simulink model "s_c_nbe_m32k"  (R2018a)
settings: Solver=VariableStepDiscrete  StartTime=0.0  StopTime=1000  RelTol=1e-3
undefined symbols (not defined in the file): fft_stages, n_taps, output_bits, pfb_coeff_gen_calc, xengbits
libraries: xbsIndex_r4 x23714, casper_library_misc x17, xps_library x4, casper_library_scopes x4, xbsReplacements_r4 x4
(part 120 of 171)

== system s_c_nbe_m32k/nb_pfb/pfb_fir_generic1/pfb_fir_coeff_gen/b_expand ==
  bus_in : Inport
  reinterpret1 : xbsIndex_r4/Reinterpret  force_arith_type=on  arith_type=Unsigned  force_bin_pt=on  bin_pt=0  block_type=reinterpret
  reinterpret2 : xbsIndex_r4/Reinterpret  force_arith_type=on  arith_type=Unsigned  force_bin_pt=on  bin_pt=0  block_type=reinterpret
  slice1 : xbsIndex_r4/Slice  nbits=18  boolean_output=off  mode=Upper Bit Location + Width  bit1=-18  base1=MSB of Input  bit0=0  base0=LSB of Input  dbl_ovrd=off  block_type=slice
  slice2 : xbsIndex_r4/Slice  nbits=18  boolean_output=off  mode=Upper Bit Location + Width  bit1=0  base1=MSB of Input  bit0=0  base0=LSB of Input  dbl_ovrd=off  block_type=slice
  msb_out2 : Outport
  lsb_out1 : Outport  Port=2
  wires:
  bus_in/1 -> slice2/1, slice1/1
  slice2/1 -> reinterpret2/1
  reinterpret2/1 -> msb_out2/1
  slice1/1 -> reinterpret1/1
  reinterpret1/1 -> lsb_out1/1

== system s_c_nbe_m32k/nb_pfb/pfb_fir_generic1/pfb_fir_coeff_gen/munge ==
  din : Inport
  join : Subsystem  AncestorBlock=casper_library_flow_control/bus_create  mask(bus_create){inputNum=2}
      mask prompts: inputNum "Number of inputs:"
      mask init:
      | bus_create_init(gcb,...
      |     'inputNum', inputNum);
  reinterpret : xbsIndex_r4/Reinterpret  force_arith_type=on  arith_type=Unsigned  force_bin_pt=on  bin_pt=0  block_type=reinterpret
  reinterpret_out : xbsIndex_r4/Reinterpret  force_arith_type=on  arith_type=Unsigned  force_bin_pt=on  bin_pt=0  block_type=reinterpret
  split : Subsystem  AncestorBlock=casper_library_flow_control/bus_expand  mask(bus_expand){mode=divisions of arbitrary size, outputNum=1, outputWidth=[18 18], outputBinaryPt=[0 0], outputArithmeticType=[0 0], show_format=off, outputToWorkspace=off, variablePrefix=out, outputToModelAsWell=on}
      mask prompts: outputNum "Number of outputs:"; outputWidth "Output width [msb ... lsb]:"; outputBinaryPt "Output binary point position [msb ... lsb]:"; outputArithmeticType "Output arithmetic type (ufix=0, fix=1, bool=2) [msb ... lsb]:"; show_format "Print format string?"; outputToWorkspace "Output to workspace?"; variablePrefix "Variable name prefix:"; outputToModelAsWell "Output to model as well?"
      mask help:
      | Expands a 'bus' made using a bus_create or Xilinx
      | concat block.
      | The input will be divided into the specified number
      | of outputs with the specified arithmetic types.
      | Divisions are made from most significant bit.
      mask init: same as s_c_nbe_m32k/bus_expand1
      settings: AttributesFormatString=2 outputs
      mask TypeOptions mode: divisions of equal size | divisions of arbitrary size
      mask Callback mode: bus_expand_callback();
      mask Callback outputWidth: bus_expand_callback();
      mask Callback outputToWorkspace: bus_expand_callback();
  dout : Outport
  wires:
  reinterpret_out/1 -> dout/1
  din/1 -> reinterpret/1
  reinterpret/1 -> split/1(bus_in)
  join/1(bus_out) -> reinterpret_out/1
  split/2(lsb_out1) -> join/1(in1)
  split/1(msb_out2) -> join/2(in2)

== system s_c_nbe_m32k/nb_pfb/pfb_fir_generic1/pfb_fir_coeff_gen/rom ==
  addra : Inport
  dina : Inport  Port=2
  wea : Inport  Port=3
  addrb : Inport  Port=4
  dinb : Inport  Port=5
  web : Inport  Port=6
  A_bussify0 : Subsystem  AncestorBlock=casper_library_flow_control/bus_create  mask(bus_create){inputNum=36}
      mask prompts: inputNum "Number of inputs:"
      mask init:
      | bus_create_init(gcb,...
      |     'inputNum', inputNum);
  B_bussify0 : Subsystem  AncestorBlock=casper_library_flow_control/bus_create  mask(bus_create){inputNum=36}
      mask prompts: inputNum "Number of inputs:"
      mask init:
      | bus_create_init(gcb,...
      |     'inputNum', inputNum);
  alsbs_slice : xbsIndex_r4/Slice  nbits=15  boolean_output=off  mode=Lower Bit Location + Width  bit1=0  base1=LSB of Input  bit0=0  base0=LSB of Input  dbl_ovrd=off  block_type=slice
  blsbs_slice : xbsIndex_r4/Slice  nbits=15  boolean_output=off  mode=Lower Bit Location + Width  bit1=0  base1=LSB of Input  bit0=0  base0=LSB of Input  dbl_ovrd=off  block_type=slice
  bram0_{0..35} (36 alike) : xbsIndex_r4/Dual Port RAM  depth=32768  initVector=getfield(get_param(gcb, 'UserData'), 'initVector')  distributed_mem=Block RAM  init_a=0  init_b=0  rst_a=off  rst_b=off  en_a=off  en_b=off  latency=7  write_mode_A=Read Before Write  write_mode_B=Read Before Write  optimize=Speed  dbl_ovrd=off  block_type=dpram
  ddina0 : xbsIndex_r4/Delay  rst=off  infoeditControl=Selection of Reset will increase slice count due to use of real FFs and instead of SRLs  en=off  latency=0  reg_retiming=on  dbl_ovrd=off  block_type=delay
  ddinb0 : xbsIndex_r4/Delay  rst=off  infoeditControl=Selection of Reset will increase slice count due to use of real FFs and instead of SRLs  en=off  latency=0  reg_retiming=on  dbl_ovrd=off  block_type=delay
  debus_addra0 : Subsystem  AncestorBlock=casper_library_flow_control/bus_expand  mask(bus_expand){mode=divisions of equal size, outputNum=36, outputWidth=[15 15 15 15 15 15 15 15 15 15 15 15 15 15 15 15 15 15 15 15 15 15 15 15 15 15 15 15 15 15 15 15 15 15 15 15], outputBinaryPt=[0 0 0 0 0 0 0 0 0 0 0 0 0 0 0 0 0 0 0 0 0 0 0 0 0 0 0 0 0 0 0 0 0 0 0 0], outputArithmeticType=[0 0 0 0 0 0 0 0 0 0 0 0 0 0 0 0 0 0 0 0 0 0 0 0 0 0 0 0 0 0 0 0 0 0 0 0], show_format=on, outputToWorkspace=off, variablePrefix=, outputToModelAsWell=on}
      mask prompts: outputNum "Number of outputs:"; outputWidth "Output width:"; outputBinaryPt "Output binary point position:"; outputArithmeticType "Output arithmetic type (ufix=0, fix=1, bool=2):"; show_format "Print format string?"; outputToWorkspace "Output to workspace?"; variablePrefix "Variable name prefix:"; outputToModelAsWell "Output to model as well?"
      mask help:
      | Expands a 'bus' made using a bus_create or Xilinx
      | concat block.
      | The input will be divided into the specified number
      | of outputs with the specified arithmetic types.
      | Divisions are made from most significant bit.
      mask init: same as s_c_nbe_m32k/bus_expand1
      settings: AttributesFormatString=36 outputs: uf15.0,uf15.0,uf15.0,uf15.0,uf15.0,uf15.0,uf15.0,uf15.0,uf15.0,uf15.0,uf15.0,uf15.0,uf15.0,uf15.0,uf15.0,uf15.0,uf15.0,uf15.0,uf15.0,uf15.0,uf15.0,uf15.0,uf15.0,uf15.0,uf15.0,uf15.0,uf15.0,uf15.0,uf15.0,uf15.0,uf15.0,uf15.0,uf15.0,uf15.0,uf15.0,uf15.0,
      mask TypeOptions mode: divisions of equal size | divisions of arbitrary size
      mask Callback mode: bus_expand_callback();
      mask Callback outputWidth: bus_expand_callback();
      mask Callback outputToWorkspace: bus_expand_callback();
  debus_addrb0 : Subsystem  AncestorBlock=casper_library_flow_control/bus_expand  mask(bus_expand){mode=divisions of equal size, outputNum=36, outputWidth=[15 15 15 15 15 15 15 15 15 15 15 15 15 15 15 15 15 15 15 15 15 15 15 15 15 15 15 15 15 15 15 15 15 15 15 15], outputBinaryPt=[0 0 0 0 0 0 0 0 0 0 0 0 0 0 0 0 0 0 0 0 0 0 0 0 0 0 0 0 0 0 0 0 0 0 0 0], outputArithmeticType=[0 0 0 0 0 0 0 0 0 0 0 0 0 0 0 0 0 0 0 0 0 0 0 0 0 0 0 0 0 0 0 0 0 0 0 0], show_format=on, outputToWorkspace=off, variablePrefix=, outputToModelAsWell=on}
      mask prompts: outputNum "Number of outputs:"; outputWidth "Output width:"; outputBinaryPt "Output binary point position:"; outputArithmeticType "Output arithmetic type (ufix=0, fix=1, bool=2):"; show_format "Print format string?"; outputToWorkspace "Output to workspace?"; variablePrefix "Variable name prefix:"; outputToModelAsWell "Output to model as well?"
      mask help:
      | Expands a 'bus' made using a bus_create or Xilinx
      | concat block.
      | The input will be divided into the specified number
      | of outputs with the specified arithmetic types.
      | Divisions are made from most significant bit.
      mask init: same as s_c_nbe_m32k/bus_expand1
      settings: AttributesFormatString=36 outputs: uf15.0,uf15.0,uf15.0,uf15.0,uf15.0,uf15.0,uf15.0,uf15.0,uf15.0,uf15.0,uf15.0,uf15.0,uf15.0,uf15.0,uf15.0,uf15.0,uf15.0,uf15.0,uf15.0,uf15.0,uf15.0,uf15.0,uf15.0,uf15.0,uf15.0,uf15.0,uf15.0,uf15.0,uf15.0,uf15.0,uf15.0,uf15.0,uf15.0,uf15.0,uf15.0,uf15.0,
      mask TypeOptions mode: divisions of equal size | divisions of arbitrary size
      mask Callback mode: bus_expand_callback();
      mask Callback outputWidth: bus_expand_callback();
      mask Callback outputToWorkspace: bus_expand_callback();
  debus_dina0 : Subsystem  AncestorBlock=casper_library_flow_control/bus_expand  mask(bus_expand){mode=divisions of arbitrary size, outputNum=1, outputWidth=[1 1 1 1 1 1 1 1 1 1 1 1 1 1 1 1 1 1 1 1 1 1 1 1 1 1 1 1 1 1 1 1 1 1 1 1], outputBinaryPt=[0 0 0 0 0 0 0 0 0 0 0 0 0 0 0 0 0 0 0 0 0 0 0 0 0 0 0 0 0 0 0 0 0 0 0 0], outputArithmeticType=[0 0 0 0 0 0 0 0 0 0 0 0 0 0 0 0 0 0 0 0 0 0 0 0 0 0 0 0 0 0 0 0 0 0 0 0], show_format=on, outputToWorkspace=off, variablePrefix=, outputToModelAsWell=on}
      mask prompts: outputNum "Number of outputs:"; outputWidth "Output width [msb ... lsb]:"; outputBinaryPt "Output binary point position [msb ... lsb]:"; outputArithmeticType "Output arithmetic type (ufix=0, fix=1, bool=2) [msb ... lsb]:"; show_format "Print format string?"; outputToWorkspace "Output to workspace?"; variablePrefix "Variable name prefix:"; outputToModelAsWell "Output to model as well?"
      mask help:
      | Expands a 'bus' made using a bus_create or Xilinx
      | concat block.
      | The input will be divided into the specified number
      | of outputs with the specified arithmetic types.
      | Divisions are made from most significant bit.
      mask init: same as s_c_nbe_m32k/bus_expand1
      settings: AttributesFormatString=36 outputs: uf1.0,uf1.0,uf1.0,uf1.0,uf1.0,uf1.0,uf1.0,uf1.0,uf1.0,uf1.0,uf1.0,uf1.0,uf1.0,uf1.0,uf1.0,uf1.0,uf1.0,uf1.0,uf1.0,uf1.0,uf1.0,uf1.0,uf1.0,uf1.0,uf1.0,uf1.0,uf1.0,uf1.0,uf1.0,uf1.0,uf1.0,uf1.0,uf1.0,uf1.0,uf1.0,uf1.0,
      mask TypeOptions mode: divisions of equal size | divisions of arbitrary size
      mask Callback mode: bus_expand_callback();
      mask Callback outputWidth: bus_expand_callback();
      mask Callback outputToWorkspace: bus_expand_callback();
  debus_dinb0 : Subsystem  AncestorBlock=casper_library_flow_control/bus_expand  mask(bus_expand){mode=divisions of arbitrary size, outputNum=1, outputWidth=[1 1 1 1 1 1 1 1 1 1 1 1 1 1 1 1 1 1 1 1 1 1 1 1 1 1 1 1 1 1 1 1 1 1 1 1], outputBinaryPt=[0 0 0 0 0 0 0 0 0 0 0 0 0 0 0 0 0 0 0 0 0 0 0 0 0 0 0 0 0 0 0 0 0 0 0 0], outputArithmeticType=[0 0 0 0 0 0 0 0 0 0 0 0 0 0 0 0 0 0 0 0 0 0 0 0 0 0 0 0 0 0 0 0 0 0 0 0], show_format=on, outputToWorkspace=off, variablePrefix=, outputToModelAsWell=on}
      mask prompts: outputNum "Number of outputs:"; outputWidth "Output width [msb ... lsb]:"; outputBinaryPt "Output binary point position [msb ... lsb]:"; outputArithmeticType "Output arithmetic type (ufix=0, fix=1, bool=2) [msb ... lsb]:"; show_format "Print format string?"; outputToWorkspace "Output to workspace?"; variablePrefix "Variable name prefix:"; outputToModelAsWell "Output to model as well?"
      mask help:
      | Expands a 'bus' made using a bus_create or Xilinx
      | concat block.
      | The input will be divided into the specified number
      | of outputs with the specified arithmetic types.
      | Divisions are made from most significant bit.
      mask init: same as s_c_nbe_m32k/bus_expand1
      settings: AttributesFormatString=36 outputs: uf1.0,uf1.0,uf1.0,uf1.0,uf1.0,uf1.0,uf1.0,uf1.0,uf1.0,uf1.0,uf1.0,uf1.0,uf1.0,uf1.0,uf1.0,uf1.0,uf1.0,uf1.0,uf1.0,uf1.0,uf1.0,uf1.0,uf1.0,uf1.0,uf1.0,uf1.0,uf1.0,uf1.0,uf1.0,uf1.0,uf1.0,uf1.0,uf1.0,uf1.0,uf1.0,uf1.0,
      mask TypeOptions mode: divisions of equal size | divisions of arbitrary size
      mask Callback mode: bus_expand_callback();
      mask Callback outputWidth: bus_expand_callback();
      mask Callback outputToWorkspace: bus_expand_callback();
  debus_wea0 : Subsystem  AncestorBlock=casper_library_flow_control/bus_expand  mask(bus_expand){mode=divisions of equal size, outputNum=36, outputWidth=[1 1 1 1 1 1 1 1 1 1 1 1 1 1 1 1 1 1 1 1 1 1 1 1 1 1 1 1 1 1 1 1 1 1 1 1], outputBinaryPt=[0 0 0 0 0 0 0 0 0 0 0 0 0 0 0 0 0 0 0 0 0 0 0 0 0 0 0 0 0 0 0 0 0 0 0 0], outputArithmeticType=[2 2 2 2 2 2 2 2 2 2 2 2 2 2 2 2 2 2 2 2 2 2 2 2 2 2 2 2 2 2 2 2 2 2 2 2], show_format=on, outputToWorkspace=off, variablePrefix=, outputToModelAsWell=on}
      mask prompts: outputNum "Number of outputs:"; outputWidth "Output width:"; outputBinaryPt "Output binary point position:"; outputArithmeticType "Output arithmetic type (ufix=0, fix=1, bool=2):"; show_format "Print format string?"; outputToWorkspace "Output to workspace?"; variablePrefix "Variable name prefix:"; outputToModelAsWell "Output to model as well?"
      mask help:
      | Expands a 'bus' made using a bus_create or Xilinx
      | concat block.
      | The input will be divided into the specified number
      | of outputs with the specified arithmetic types.
      | Divisions are made from most significant bit.
      mask init: same as s_c_nbe_m32k/bus_expand1
      settings: AttributesFormatString=36 outputs: b,b,b,b,b,b,b,b,b,b,b,b,b,b,b,b,b,b,b,b,b,b,b,b,b,b,b,b,b,b,b,b,b,b,b,b,
      mask TypeOptions mode: divisions of equal size | divisions of arbitrary size
      mask Callback mode: bus_expand_callback();
      mask Callback outputWidth: bus_expand_callback();
      mask Callback outputToWorkspace: bus_expand_callback();
  debus_web0 : Subsystem  AncestorBlock=casper_library_flow_control/bus_expand  mask(bus_expand){mode=divisions of equal size, outputNum=36, outputWidth=[1 1 1 1 1 1 1 1 1 1 1 1 1 1 1 1 1 1 1 1 1 1 1 1 1 1 1 1 1 1 1 1 1 1 1 1], outputBinaryPt=[0 0 0 0 0 0 0 0 0 0 0 0 0 0 0 0 0 0 0 0 0 0 0 0 0 0 0 0 0 0 0 0 0 0 0 0], outputArithmeticType=[2 2 2 2 2 2 2 2 2 2 2 2 2 2 2 2 2 2 2 2 2 2 2 2 2 2 2 2 2 2 2 2 2 2 2 2], show_format=on, outputToWorkspace=off, variablePrefix=, outputToModelAsWell=on}
      mask prompts: outputNum "Number of outputs:"; outputWidth "Output width:"; outputBinaryPt "Output binary point position:"; outputArithmeticType "Output arithmetic type (ufix=0, fix=1, bool=2):"; show_format "Print format string?"; outputToWorkspace "Output to workspace?"; variablePrefix "Variable name prefix:"; outputToModelAsWell "Output to model as well?"
      mask help:
      | Expands a 'bus' made using a bus_create or Xilinx
      | concat block.
      | The input will be divided into the specified number
      | of outputs with the specified arithmetic types.
      | Divisions are made from most significant bit.
      mask init: same as s_c_nbe_m32k/bus_expand1
      settings: AttributesFormatString=36 outputs: b,b,b,b,b,b,b,b,b,b,b,b,b,b,b,b,b,b,b,b,b,b,b,b,b,b,b,b,b,b,b,b,b,b,b,b,
      mask TypeOptions mode: divisions of equal size | divisions of arbitrary size
      mask Callback mode: bus_expand_callback();
      mask Callback outputWidth: bus_expand_callback();
      mask Callback outputToWorkspace: bus_expand_callback();
  rep_addra0 : Subsystem  AncestorBlock=casper_library_bus/bus_replicate  mask(bus_replicate){replication=36, csp_latency=4, misc=off, implementation=core}
      mask prompts: replication "replication factor"; csp_latency "latency"; misc "misc support"; implementation "delay implementation"
      mask help: Output bus formed by replicating input bus a number of times
      mask init:
      | bus_replicate_init(gcb, ...
      |     'replication', replication, ...
      |     'csp_latency', csp_latency, ...
      |     'implementation', implementation, ...
      |     'misc', misc);
      mask TypeOptions implementation: core | behavioral
  rep_addrb0 : Subsystem  AncestorBlock=casper_library_bus/bus_replicate  mask(bus_replicate){replication=36, csp_latency=4, misc=off, implementation=core}
      mask prompts: replication "replication factor"; csp_latency "latency"; misc "misc support"; implementation "delay implementation"
      mask help: Output bus formed by replicating input bus a number of times
      mask init:
      | bus_replicate_init(gcb, ...
      |     'replication', replication, ...
      |     'csp_latency', csp_latency, ...
      |     'implementation', implementation, ...
      |     'misc', misc);
      mask TypeOptions implementation: core | behavioral
  rep_wea0 : Subsystem  AncestorBlock=casper_library_bus/bus_replicate  mask(bus_replicate){replication=36, csp_latency=0, misc=off, implementation=behavioral}
      mask prompts: replication "replication factor"; csp_latency "latency"; misc "misc support"; implementation "delay implementation"
      mask help: Output bus formed by replicating input bus a number of times
      mask init:
      | bus_replicate_init(gcb, ...
      |     'replication', replication, ...
      |     'csp_latency', csp_latency, ...
      |     'implementation', implementation, ...
      |     'misc', misc);
      mask TypeOptions implementation: core | behavioral
  rep_web0 : Subsystem  AncestorBlock=casper_library_bus/bus_replicate  mask(bus_replicate){replication=36, csp_latency=0, misc=off, implementation=behavioral}
      mask prompts: replication "replication factor"; csp_latency "latency"; misc "misc support"; implementation "delay implementation"
      mask help: Output bus formed by replicating input bus a number of times
      mask init:
      | bus_replicate_init(gcb, ...
      |     'replication', replication, ...
      |     'csp_latency', csp_latency, ...
      |     'implementation', implementation, ...
      |     'misc', misc);
      mask TypeOptions implementation: core | behavioral
  A : Outport
  B : Outport  Port=2
  wires:
  addrb/1 -> blsbs_slice/1
  addra/1 -> alsbs_slice/1
  blsbs_slice/1 -> rep_addrb0/1(in)
  alsbs_slice/1 -> rep_addra0/1(in)
  dina/1 -> ddina0/1
  wea/1 -> rep_wea0/1(in)
  dinb/1 -> ddinb0/1
  web/1 -> rep_web0/1(in)
  rep_addrb0/1(out) -> debus_addrb0/1(bus_in)
  rep_addra0/1(out) -> debus_addra0/1(bus_in)
  ddina0/1 -> debus_dina0/1(bus_in)
  rep_wea0/1(out) -> debus_wea0/1(bus_in)
  ddinb0/1 -> debus_dinb0/1(bus_in)
  rep_web0/1(out) -> debus_web0/1(bus_in)
  debus_addra0/1(msb_out36) -> bram0_0/1
  debus_dina0/1(msb_out36) -> bram0_0/2
  debus_wea0/1(msb_out36) -> bram0_0/3
  debus_addrb0/1(msb_out36) -> bram0_0/4
  debus_dinb0/1(msb_out36) -> bram0_0/5
  debus_web0/1(msb_out36) -> bram0_0/6
  debus_addra0/2(out35) -> bram0_1/1
  debus_dina0/2(out35) -> bram0_1/2
  debus_wea0/2(out35) -> bram0_1/3
  debus_addrb0/2(out35) -> bram0_1/4
  debus_dinb0/2(out35) -> bram0_1/5
  debus_web0/2(out35) -> bram0_1/6
  debus_addra0/3(out34) -> bram0_2/1
  debus_dina0/3(out34) -> bram0_2/2
  debus_wea0/3(out34) -> bram0_2/3
  debus_addrb0/3(out34) -> bram0_2/4
  debus_dinb0/3(out34) -> bram0_2/5
  debus_web0/3(out34) -> bram0_2/6
  debus_addra0/4(out33) -> bram0_3/1
  debus_dina0/4(out33) -> bram0_3/2
  debus_wea0/4(out33) -> bram0_3/3
  debus_addrb0/4(out33) -> bram0_3/4
  debus_dinb0/4(out33) -> bram0_3/5
  debus_web0/4(out33) -> bram0_3/6
  debus_addra0/5(out32) -> bram0_4/1
  debus_dina0/5(out32) -> bram0_4/2
  debus_wea0/5(out32) -> bram0_4/3
  debus_addrb0/5(out32) -> bram0_4/4
  debus_dinb0/5(out32) -> bram0_4/5
  debus_web0/5(out32) -> bram0_4/6
  debus_addra0/6(out31) -> bram0_5/1
  debus_dina0/6(out31) -> bram0_5/2
  debus_wea0/6(out31) -> bram0_5/3
  debus_addrb0/6(out31) -> bram0_5/4
  debus_dinb0/6(out31) -> bram0_5/5
  debus_web0/6(out31) -> bram0_5/6
  debus_addra0/7(out30) -> bram0_6/1
  debus_dina0/7(out30) -> bram0_6/2
  debus_wea0/7(out30) -> bram0_6/3
  debus_addrb0/7(out30) -> bram0_6/4
  debus_dinb0/7(out30) -> bram0_6/5
  debus_web0/7(out30) -> bram0_6/6
  debus_addra0/8(out29) -> bram0_7/1
  debus_dina0/8(out29) -> bram0_7/2
  debus_wea0/8(out29) -> bram0_7/3
  debus_addrb0/8(out29) -> bram0_7/4
  debus_dinb0/8(out29) -> bram0_7/5
  debus_web0/8(out29) -> bram0_7/6
  debus_addra0/9(out28) -> bram0_8/1
  debus_dina0/9(out28) -> bram0_8/2
  debus_wea0/9(out28) -> bram0_8/3
  debus_addrb0/9(out28) -> bram0_8/4
  debus_dinb0/9(out28) -> bram0_8/5
  debus_web0/9(out28) -> bram0_8/6
  debus_addra0/10(out27) -> bram0_9/1
  debus_dina0/10(out27) -> bram0_9/2
  debus_wea0/10(out27) -> bram0_9/3
  debus_addrb0/10(out27) -> bram0_9/4
  debus_dinb0/10(out27) -> bram0_9/5
  debus_web0/10(out27) -> bram0_9/6
  debus_addra0/11(out26) -> bram0_10/1
  debus_dina0/11(out26) -> bram0_10/2
  debus_wea0/11(out26) -> bram0_10/3
  debus_addrb0/11(out26) -> bram0_10/4
  debus_dinb0/11(out26) -> bram0_10/5
  debus_web0/11(out26) -> bram0_10/6
  debus_addra0/12(out25) -> bram0_11/1
  debus_dina0/12(out25) -> bram0_11/2
  debus_wea0/12(out25) -> bram0_11/3
  debus_addrb0/12(out25) -> bram0_11/4
  debus_dinb0/12(out25) -> bram0_11/5
  debus_web0/12(out25) -> bram0_11/6
  debus_addra0/13(out24) -> bram0_12/1
  debus_dina0/13(out24) -> bram0_12/2
  debus_wea0/13(out24) -> bram0_12/3
  debus_addrb0/13(out24) -> bram0_12/4
  debus_dinb0/13(out24) -> bram0_12/5
  debus_web0/13(out24) -> bram0_12/6
  debus_addra0/14(out23) -> bram0_13/1
  debus_dina0/14(out23) -> bram0_13/2
  debus_wea0/14(out23) -> bram0_13/3
  debus_addrb0/14(out23) -> bram0_13/4
  debus_dinb0/14(out23) -> bram0_13/5
  debus_web0/14(out23) -> bram0_13/6
  debus_addra0/15(out22) -> bram0_14/1
  debus_dina0/15(out22) -> bram0_14/2
  debus_wea0/15(out22) -> bram0_14/3
  debus_addrb0/15(out22) -> bram0_14/4
  debus_dinb0/15(out22) -> bram0_14/5
  debus_web0/15(out22) -> bram0_14/6
  debus_addra0/16(out21) -> bram0_15/1
  debus_dina0/16(out21) -> bram0_15/2
  debus_wea0/16(out21) -> bram0_15/3
  debus_addrb0/16(out21) -> bram0_15/4
  debus_dinb0/16(out21) -> bram0_15/5
  debus_web0/16(out21) -> bram0_15/6
  debus_addra0/17(out20) -> bram0_16/1
  debus_dina0/17(out20) -> bram0_16/2
  debus_wea0/17(out20) -> bram0_16/3
  debus_addrb0/17(out20) -> bram0_16/4
  debus_dinb0/17(out20) -> bram0_16/5
  debus_web0/17(out20) -> bram0_16/6
  debus_addra0/18(out19) -> bram0_17/1
  debus_dina0/18(out19) -> bram0_17/2
  debus_wea0/18(out19) -> bram0_17/3
  debus_addrb0/18(out19) -> bram0_17/4
  debus_dinb0/18(out19) -> bram0_17/5
  debus_web0/18(out19) -> bram0_17/6
  debus_addra0/19(out18) -> bram0_18/1
  debus_dina0/19(out18) -> bram0_18/2
  debus_wea0/19(out18) -> bram0_18/3
  debus_addrb0/19(out18) -> bram0_18/4
  debus_dinb0/19(out18) -> bram0_18/5
  debus_web0/19(out18) -> bram0_18/6
  debus_addra0/20(out17) -> bram0_19/1
  debus_dina0/20(out17) -> bram0_19/2
  debus_wea0/20(out17) -> bram0_19/3
  debus_addrb0/20(out17) -> bram0_19/4
  debus_dinb0/20(out17) -> bram0_19/5
  debus_web0/20(out17) -> bram0_19/6
  debus_addra0/21(out16) -> bram0_20/1
  debus_dina0/21(out16) -> bram0_20/2
  debus_wea0/21(out16) -> bram0_20/3
  debus_addrb0/21(out16) -> bram0_20/4
  debus_dinb0/21(out16) -> bram0_20/5
  debus_web0/21(out16) -> bram0_20/6
  debus_addra0/22(out15) -> bram0_21/1
  debus_dina0/22(out15) -> bram0_21/2
  debus_wea0/22(out15) -> bram0_21/3
  debus_addrb0/22(out15) -> bram0_21/4
  debus_dinb0/22(out15) -> bram0_21/5
  debus_web0/22(out15) -> bram0_21/6
  debus_addra0/23(out14) -> bram0_22/1
  debus_dina0/23(out14) -> bram0_22/2
  debus_wea0/23(out14) -> bram0_22/3
  debus_addrb0/23(out14) -> bram0_22/4
  debus_dinb0/23(out14) -> bram0_22/5
  debus_web0/23(out14) -> bram0_22/6
  debus_addra0/24(out13) -> bram0_23/1
  debus_dina0/24(out13) -> bram0_23/2
  debus_wea0/24(out13) -> bram0_23/3
  debus_addrb0/24(out13) -> bram0_23/4
  debus_dinb0/24(out13) -> bram0_23/5
  debus_web0/24(out13) -> bram0_23/6
  debus_addra0/25(out12) -> bram0_24/1
  debus_dina0/25(out12) -> bram0_24/2
  debus_wea0/25(out12) -> bram0_24/3
  debus_addrb0/25(out12) -> bram0_24/4
  debus_dinb0/25(out12) -> bram0_24/5
  debus_web0/25(out12) -> bram0_24/6
  debus_addra0/26(out11) -> bram0_25/1
  debus_dina0/26(out11) -> bram0_25/2
  debus_wea0/26(out11) -> bram0_25/3
  debus_addrb0/26(out11) -> bram0_25/4
  debus_dinb0/26(out11) -> bram0_25/5
  debus_web0/26(out11) -> bram0_25/6
  debus_addra0/27(out10) -> bram0_26/1
  debus_dina0/27(out10) -> bram0_26/2
  debus_wea0/27(out10) -> bram0_26/3
  debus_addrb0/27(out10) -> bram0_26/4
  debus_dinb0/27(out10) -> bram0_26/5
  debus_web0/27(out10) -> bram0_26/6
  debus_addra0/28(out9) -> bram0_27/1
  debus_dina0/28(out9) -> bram0_27/2
  debus_wea0/28(out9) -> bram0_27/3
  debus_addrb0/28(out9) -> bram0_27/4
  debus_dinb0/28(out9) -> bram0_27/5
  debus_web0/28(out9) -> bram0_27/6
  debus_addra0/29(out8) -> bram0_28/1
  debus_dina0/29(out8) -> bram0_28/2
  debus_wea0/29(out8) -> bram0_28/3
  debus_addrb0/29(out8) -> bram0_28/4
  debus_dinb0/29(out8) -> bram0_28/5
  debus_web0/29(out8) -> bram0_28/6
  debus_addra0/30(out7) -> bram0_29/1
  debus_dina0/30(out7) -> bram0_29/2
  debus_wea0/30(out7) -> bram0_29/3
  debus_addrb0/30(out7) -> bram0_29/4
  debus_dinb0/30(out7) -> bram0_29/5
  debus_web0/30(out7) -> bram0_29/6
  debus_addra0/31(out6) -> bram0_30/1
  debus_dina0/31(out6) -> bram0_30/2
  debus_wea0/31(out6) -> bram0_30/3
  debus_addrb0/31(out6) -> bram0_30/4
  debus_dinb0/31(out6) -> bram0_30/5
  debus_web0/31(out6) -> bram0_30/6
  debus_addra0/32(out5) -> bram0_31/1
  debus_dina0/32(out5) -> bram0_31/2
  debus_wea0/32(out5) -> bram0_31/3
  debus_addrb0/32(out5) -> bram0_31/4
  debus_dinb0/32(out5) -> bram0_31/5
  debus_web0/32(out5) -> bram0_31/6
  debus_addra0/33(out4) -> bram0_32/1
  debus_dina0/33(out4) -> bram0_32/2
  debus_wea0/33(out4) -> bram0_32/3
  debus_addrb0/33(out4) -> bram0_32/4
  debus_dinb0/33(out4) -> bram0_32/5
  debus_web0/33(out4) -> bram0_32/6
  debus_addra0/34(out3) -> bram0_33/1
  debus_dina0/34(out3) -> bram0_33/2
  debus_wea0/34(out3) -> bram0_33/3
  debus_addrb0/34(out3) -> bram0_33/4
  debus_dinb0/34(out3) -> bram0_33/5
  debus_web0/34(out3) -> bram0_33/6
  debus_addra0/35(out2) -> bram0_34/1
  debus_dina0/35(out2) -> bram0_34/2
  debus_wea0/35(out2) -> bram0_34/3
  debus_addrb0/35(out2) -> bram0_34/4
  debus_dinb0/35(out2) -> bram0_34/5
  debus_web0/35(out2) -> bram0_34/6
  debus_addra0/36(lsb_out1) -> bram0_35/1
  debus_dina0/36(lsb_out1) -> bram0_35/2
  debus_wea0/36(lsb_out1) -> bram0_35/3
  debus_addrb0/36(lsb_out1) -> bram0_35/4
  debus_dinb0/36(lsb_out1) -> bram0_35/5
  debus_web0/36(lsb_out1) -> bram0_35/6
  bram0_0/1 -> A_bussify0/1(in1)
  bram0_0/2 -> B_bussify0/1(in1)
  bram0_1/1 -> A_bussify0/2(in2)
  bram0_1/2 -> B_bussify0/2(in2)
  bram0_2/1 -> A_bussify0/3(in3)
  bram0_2/2 -> B_bussify0/3(in3)
  bram0_3/1 -> A_bussify0/4(in4)
  bram0_3/2 -> B_bussify0/4(in4)
  bram0_4/1 -> A_bussify0/5(in5)
  bram0_4/2 -> B_bussify0/5(in5)
  bram0_5/1 -> A_bussify0/6(in6)
  bram0_5/2 -> B_bussify0/6(in6)
  bram0_6/1 -> A_bussify0/7(in7)
  bram0_6/2 -> B_bussify0/7(in7)
  bram0_7/1 -> A_bussify0/8(in8)
  bram0_7/2 -> B_bussify0/8(in8)
  bram0_8/1 -> A_bussify0/9(in9)
  bram0_8/2 -> B_bussify0/9(in9)
  bram0_9/1 -> A_bussify0/10(in10)
  bram0_9/2 -> B_bussify0/10(in10)
  bram0_10/1 -> A_bussify0/11(in11)
  bram0_10/2 -> B_bussify0/11(in11)
  bram0_11/1 -> A_bussify0/12(in12)
  bram0_11/2 -> B_bussify0/12(in12)
  bram0_12/1 -> A_bussify0/13(in13)
  bram0_12/2 -> B_bussify0/13(in13)
  bram0_13/1 -> A_bussify0/14(in14)
  bram0_13/2 -> B_bussify0/14(in14)
  bram0_14/1 -> A_bussify0/15(in15)
  bram0_14/2 -> B_bussify0/15(in15)
  bram0_15/1 -> A_bussify0/16(in16)
  bram0_15/2 -> B_bussify0/16(in16)
  bram0_16/1 -> A_bussify0/17(in17)
  bram0_16/2 -> B_bussify0/17(in17)
  bram0_17/1 -> A_bussify0/18(in18)
  bram0_17/2 -> B_bussify0/18(in18)
  bram0_18/1 -> A_bussify0/19(in19)
  bram0_18/2 -> B_bussify0/19(in19)
  bram0_19/1 -> A_bussify0/20(in20)
  bram0_19/2 -> B_bussify0/20(in20)
  bram0_20/1 -> A_bussify0/21(in21)
  bram0_20/2 -> B_bussify0/21(in21)
  bram0_21/1 -> A_bussify0/22(in22)
  bram0_21/2 -> B_bussify0/22(in22)
  bram0_22/1 -> A_bussify0/23(in23)
  bram0_22/2 -> B_bussify0/23(in23)
  bram0_23/1 -> A_bussify0/24(in24)
  bram0_23/2 -> B_bussify0/24(in24)
  bram0_24/1 -> A_bussify0/25(in25)
  bram0_24/2 -> B_bussify0/25(in25)
  bram0_25/1 -> A_bussify0/26(in26)
  bram0_25/2 -> B_bussify0/26(in26)
  bram0_26/1 -> A_bussify0/27(in27)
  bram0_26/2 -> B_bussify0/27(in27)
  bram0_27/1 -> A_bussify0/28(in28)
  bram0_27/2 -> B_bussify0/28(in28)
  bram0_28/1 -> A_bussify0/29(in29)
  bram0_28/2 -> B_bussify0/29(in29)
  bram0_29/1 -> A_bussify0/30(in30)
  bram0_29/2 -> B_bussify0/30(in30)
  bram0_30/1 -> A_bussify0/31(in31)
  bram0_30/2 -> B_bussify0/31(in31)
  bram0_31/1 -> A_bussify0/32(in32)
  bram0_31/2 -> B_bussify0/32(in32)
  bram0_32/1 -> A_bussify0/33(in33)
  bram0_32/2 -> B_bussify0/33(in33)
  bram0_33/1 -> A_bussify0/34(in34)
  bram0_33/2 -> B_bussify0/34(in34)
  bram0_34/1 -> A_bussify0/35(in35)
  bram0_34/2 -> B_bussify0/35(in35)
  bram0_35/1 -> A_bussify0/36(in36)
  bram0_35/2 -> B_bussify0/36(in36)
  A_bussify0/1(bus_out) -> A/1
  B_bussify0/1(bus_out) -> B/1

== system s_c_nbe_m32k/nb_pfb/pfb_fir_generic1/pfb_fir_taps/bus_adder_tree ==
  d0 : Inport
  d1 : Inport  Port=2
  d2 : Inport  Port=3
  d3 : Inport  Port=4
  add_tree0 : Subsystem  mask(adder_tree){n_inputs=4, csp_latency=7, adder_imp=Behavioral, first_stage_hdl=on, floating_point=off, float_type=single, frac_width=0, exp_width=0}
      mask prompts: n_inputs "Number of Inputs"; csp_latency "Add Latency"; adder_imp "Adder implementation"; first_stage_hdl "Use behavioural HDL for first stage of adders"; floating_point "floating point"; float_type "float type"; frac_width "fraction length"; exp_width "exponent length"
      mask help:
      | Sums all inputs using a tree of adds and delays.
      |
      | Number of inputs: The number of inputs to the block to be summed
      | Add latency: The number of clock cycles to perform one addition (affects timing)..
      | Adder implementation: choice of fabric or DSP48E core, or behavioral HDL
      | Use behavioural HDL for first stage of adders: Causes the first stage of adders to be absorbed into DSP blocks if multipliers precede them (Virtex 5). Overrides Adder implementation
      mask init: same as s_c_nbe_m32k/DDC/dec_fir_async1/imag_sum
      settings: AttributesFormatString=latency 14
      mask Help: eval('xlWeb(''http://casper.berkeley.edu/wiki/Adder_tree'')')
      mask TypeOptions adder_imp: Behavioral | Fabric | DSP48
      mask Callback floating_point:
      | onoff = get_param(gcb, 'floating_point');
      | if strcmp(onoff,'on')
      |     enable_fixpt = 'off'
      |     set_param_state(gcb, 'float_type', 'on')
      | 
      |     f_type = get_param(gcb, 'float_type')
      |     if strcmp(f_type,'custom')
      |         set_param_state(gcb, 'exp_width', 'on')
      |         set_param_state(gcb, 'frac_width', 'on')
      |     else
      |         set_param_state(gcb, 'exp_width', 'off')
      |         set_param_state(gcb, 'frac_width', 'off')
      |     end
      | 
      | 
      | else
      |     enable_fixpt = 'on'
      |     set_param_state(gcb, 'float_type', 'off')
      |     set_param_state(gcb, 'exp_width', 'off')
      |     set_param_state(gcb, 'frac_width', 'off')
      | end
      mask TypeOptions float_type: single | custom
      mask Callback float_type:
      | f_type = get_param(gcb, 'float_type')
      | if strcmp(f_type,'custom')
      |     set_param_state(gcb, 'exp_width', 'on')
      |     set_param_state(gcb, 'frac_width', 'on')
      | else
      |     set_param_state(gcb, 'exp_width', 'off')
      |     set_param_state(gcb, 'frac_width', 'off')
      | end
  add_tree1 : Subsystem  mask(adder_tree){n_inputs=4, csp_latency=7, adder_imp=Behavioral, first_stage_hdl=on, floating_point=off, float_type=single, frac_width=0, exp_width=0}
      mask prompts: n_inputs "Number of Inputs"; csp_latency "Add Latency"; adder_imp "Adder implementation"; first_stage_hdl "Use behavioural HDL for first stage of adders"; floating_point "floating point"; float_type "float type"; frac_width "fraction length"; exp_width "exponent length"
      mask help:
      | Sums all inputs using a tree of adds and delays.
      |
      | Number of inputs: The number of inputs to the block to be summed
      | Add latency: The number of clock cycles to perform one addition (affects timing)..
      | Adder implementation: choice of fabric or DSP48E core, or behavioral HDL
      | Use behavioural HDL for first stage of adders: Causes the first stage of adders to be absorbed into DSP blocks if multipliers precede them (Virtex 5). Overrides Adder implementation
      mask init: same as s_c_nbe_m32k/DDC/dec_fir_async1/imag_sum
      settings: AttributesFormatString=latency 14
      mask Help: eval('xlWeb(''http://casper.berkeley.edu/wiki/Adder_tree'')')
      mask TypeOptions adder_imp: Behavioral | Fabric | DSP48
      mask Callback floating_point:
      | onoff = get_param(gcb, 'floating_point');
      | if strcmp(onoff,'on')
      |     enable_fixpt = 'off'
      |     set_param_state(gcb, 'float_type', 'on')
      | 
      |     f_type = get_param(gcb, 'float_type')
      |     if strcmp(f_type,'custom')
      |         set_param_state(gcb, 'exp_width', 'on')
      |         set_param_state(gcb, 'frac_width', 'on')
      |     else
      |         set_param_state(gcb, 'exp_width', 'off')
      |         set_param_state(gcb, 'frac_width', 'off')
      |     end
      | 
      | 
      | else
      |     enable_fixpt = 'on'
      |     set_param_state(gcb, 'float_type', 'off')
      |     set_param_state(gcb, 'exp_width', 'off')
      |     set_param_state(gcb, 'frac_width', 'off')
      | end
      mask TypeOptions float_type: single | custom
      mask Callback float_type:
      | f_type = get_param(gcb, 'float_type')
      | if strcmp(f_type,'custom')
      |     set_param_state(gcb, 'exp_width', 'on')
      |     set_param_state(gcb, 'frac_width', 'on')
      | else
      |     set_param_state(gcb, 'exp_width', 'off')
      |     set_param_state(gcb, 'frac_width', 'off')
      | end
  constant : xbsIndex_r4/Constant  const=0  gui_display_data_type=Fixed-point  arith_type=Boolean  n_bits=16  bin_pt=14  preci_type=Single  exp_width=8  frac_width=24  explicit_period=on  period=1  equ=P=C  opselect=C  inp2=PCIN>>17  opr=+  inp1=P  carry=CIN  dbl_ovrd=off  block_type=constant
  d_bussify : Subsystem  mask(bus_create){inputNum=2}
      mask prompts: inputNum "Number of inputs:"
      mask init:
      | bus_create_init(gcb,...
      |     'inputNum', inputNum);
  expand0 : Subsystem  mask(bus_expand){mode=divisions of arbitrary size, outputNum=1, outputWidth=[36 36], outputBinaryPt=[34 34], outputArithmeticType=[1 1], show_format=on, outputToWorkspace=off, variablePrefix=, outputToModelAsWell=on}
      mask prompts: outputNum "Number of outputs:"; outputWidth "Output width [msb ... lsb]:"; outputBinaryPt "Output binary point position [msb ... lsb]:"; outputArithmeticType "Output arithmetic type (ufix=0, fix=1, bool=2) [msb ... lsb]:"; show_format "Print format string?"; outputToWorkspace "Output to workspace?"; variablePrefix "Variable name prefix:"; outputToModelAsWell "Output to model as well?"
      mask help:
      | Expands a 'bus' made using a bus_create or Xilinx
      | concat block.
      | The input will be divided into the specified number
      | of outputs with the specified arithmetic types.
      | Divisions are made from most significant bit.
      mask init: same as s_c_nbe_m32k/bus_expand1
      settings: AttributesFormatString=2 outputs: f36.34,f36.34,
      mask TypeOptions mode: divisions of equal size | divisions of arbitrary size
      mask Callback mode: bus_expand_callback();
      mask Callback outputWidth: bus_expand_callback();
      mask Callback outputToWorkspace: bus_expand_callback();
  expand1 : Subsystem  mask(bus_expand){mode=divisions of arbitrary size, outputNum=1, outputWidth=[36 36], outputBinaryPt=[34 34], outputArithmeticType=[1 1], show_format=on, outputToWorkspace=off, variablePrefix=, outputToModelAsWell=on}
      mask prompts: outputNum "Number of outputs:"; outputWidth "Output width [msb ... lsb]:"; outputBinaryPt "Output binary point position [msb ... lsb]:"; outputArithmeticType "Output arithmetic type (ufix=0, fix=1, bool=2) [msb ... lsb]:"; show_format "Print format string?"; outputToWorkspace "Output to workspace?"; variablePrefix "Variable name prefix:"; outputToModelAsWell "Output to model as well?"
      mask help:
      | Expands a 'bus' made using a bus_create or Xilinx
      | concat block.
      | The input will be divided into the specified number
      | of outputs with the specified arithmetic types.
      | Divisions are made from most significant bit.
      mask init: same as s_c_nbe_m32k/bus_expand1
      settings: AttributesFormatString=2 outputs: f36.34,f36.34,
      mask TypeOptions mode: divisions of equal size | divisions of arbitrary size
      mask Callback mode: bus_expand_callback();
      mask Callback outputWidth: bus_expand_callback();
      mask Callback outputToWorkspace: bus_expand_callback();
  expand2 : Subsystem  mask(bus_expand){mode=divisions of arbitrary size, outputNum=1, outputWidth=[36 36], outputBinaryPt=[34 34], outputArithmeticType=[1 1], show_format=on, outputToWorkspace=off, variablePrefix=, outputToModelAsWell=on}
      mask prompts: outputNum "Number of outputs:"; outputWidth "Output width [msb ... lsb]:"; outputBinaryPt "Output binary point position [msb ... lsb]:"; outputArithmeticType "Output arithmetic type (ufix=0, fix=1, bool=2) [msb ... lsb]:"; show_format "Print format string?"; outputToWorkspace "Output to workspace?"; variablePrefix "Variable name prefix:"; outputToModelAsWell "Output to model as well?"
      mask help:
      | Expands a 'bus' made using a bus_create or Xilinx
      | concat block.
      | The input will be divided into the specified number
      | of outputs with the specified arithmetic types.
      | Divisions are made from most significant bit.
      mask init: same as s_c_nbe_m32k/bus_expand1
      settings: AttributesFormatString=2 outputs: f36.34,f36.34,
      mask TypeOptions mode: divisions of equal size | divisions of arbitrary size
      mask Callback mode: bus_expand_callback();
      mask Callback outputWidth: bus_expand_callback();
      mask Callback outputToWorkspace: bus_expand_callback();
  expand3 : Subsystem  mask(bus_expand){mode=divisions of arbitrary size, outputNum=1, outputWidth=[36 36], outputBinaryPt=[34 34], outputArithmeticType=[1 1], show_format=on, outputToWorkspace=off, variablePrefix=, outputToModelAsWell=on}
      mask prompts: outputNum "Number of outputs:"; outputWidth "Output width [msb ... lsb]:"; outputBinaryPt "Output binary point position [msb ... lsb]:"; outputArithmeticType "Output arithmetic type (ufix=0, fix=1, bool=2) [msb ... lsb]:"; show_format "Print format string?"; outputToWorkspace "Output to workspace?"; variablePrefix "Variable name prefix:"; outputToModelAsWell "Output to model as well?"
      mask help:
      | Expands a 'bus' made using a bus_create or Xilinx
      | concat block.
      | The input will be divided into the specified number
      | of outputs with the specified arithmetic types.
      | Divisions are made from most significant bit.
      mask init: same as s_c_nbe_m32k/bus_expand1
      settings: AttributesFormatString=2 outputs: f36.34,f36.34,
      mask TypeOptions mode: divisions of equal size | divisions of arbitrary size
      mask Callback mode: bus_expand_callback();
      mask Callback outputWidth: bus_expand_callback();
      mask Callback outputToWorkspace: bus_expand_callback();
  out : Outport
  wires:
  d0/1 -> expand0/1(bus_in)
  d1/1 -> expand1/1(bus_in)
  d2/1 -> expand2/1(bus_in)
  d3/1 -> expand3/1(bus_in)
  constant/1 -> add_tree0/1(sync), add_tree1/1(sync)
  expand0/1(msb_out2) -> add_tree0/2(din1)
  expand1/1(msb_out2) -> add_tree0/3(din2)
  expand2/1(msb_out2) -> add_tree0/4(din3)
  expand3/1(msb_out2) -> add_tree0/5(din4)
  expand0/2(lsb_out1) -> add_tree1/2(din1)
  expand1/2(lsb_out1) -> add_tree1/3(din2)
  expand2/2(lsb_out1) -> add_tree1/4(din3)
  expand3/2(lsb_out1) -> add_tree1/5(din4)
  add_tree0/2(dout) -> d_bussify/1(in1)
  add_tree1/2(dout) -> d_bussify/2(in2)
  d_bussify/1(bus_out) -> out/1

== system s_c_nbe_m32k/nb_pfb/pfb_fir_generic1/pfb_fir_taps/bus_mult ==
  a : Inport
  b : Inport  Port=2
  a*b_bussify : Subsystem  mask(bus_create){inputNum=8}
      mask prompts: inputNum "Number of inputs:"
      mask init:
      | bus_create_init(gcb,...
      |     'inputNum', inputNum);
  a_debus : Subsystem  mask(bus_expand){mode=divisions of arbitrary size, outputNum=1, outputWidth=[18 18 18 18 18 18 18 18], outputBinaryPt=[17 17 17 17 17 17 17 17], outputArithmeticType=[1 1 1 1 1 1 1 1], show_format=on, outputToWorkspace=off, variablePrefix=, outputToModelAsWell=on}
      mask prompts: outputNum "Number of outputs:"; outputWidth "Output width [msb ... lsb]:"; outputBinaryPt "Output binary point position [msb ... lsb]:"; outputArithmeticType "Output arithmetic type (ufix=0, fix=1, bool=2) [msb ... lsb]:"; show_format "Print format string?"; outputToWorkspace "Output to workspace?"; variablePrefix "Variable name prefix:"; outputToModelAsWell "Output to model as well?"
      mask help:
      | Expands a 'bus' made using a bus_create or Xilinx
      | concat block.
      | The input will be divided into the specified number
      | of outputs with the specified arithmetic types.
      | Divisions are made from most significant bit.
      mask init: same as s_c_nbe_m32k/bus_expand1
      settings: AttributesFormatString=8 outputs: f18.17,f18.17,f18.17,f18.17,f18.17,f18.17,f18.17,f18.17,
      mask TypeOptions mode: divisions of equal size | divisions of arbitrary size
      mask Callback mode: bus_expand_callback();
      mask Callback outputWidth: bus_expand_callback();
      mask Callback outputToWorkspace: bus_expand_callback();
  b_debus : Subsystem  mask(bus_expand){mode=divisions of arbitrary size, outputNum=1, outputWidth=[18 18 18 18 18 18 18 18], outputBinaryPt=[17 17 17 17 17 17 17 17], outputArithmeticType=[1 1 1 1 1 1 1 1], show_format=on, outputToWorkspace=off, variablePrefix=, outputToModelAsWell=on}
      mask prompts: outputNum "Number of outputs:"; outputWidth "Output width [msb ... lsb]:"; outputBinaryPt "Output binary point position [msb ... lsb]:"; outputArithmeticType "Output arithmetic type (ufix=0, fix=1, bool=2) [msb ... lsb]:"; show_format "Print format string?"; outputToWorkspace "Output to workspace?"; variablePrefix "Variable name prefix:"; outputToModelAsWell "Output to model as well?"
      mask help:
      | Expands a 'bus' made using a bus_create or Xilinx
      | concat block.
      | The input will be divided into the specified number
      | of outputs with the specified arithmetic types.
      | Divisions are made from most significant bit.
      mask init: same as s_c_nbe_m32k/bus_expand1
      settings: AttributesFormatString=8 outputs: f18.17,f18.17,f18.17,f18.17,f18.17,f18.17,f18.17,f18.17,
      mask TypeOptions mode: divisions of equal size | divisions of arbitrary size
      mask Callback mode: bus_expand_callback();
      mask Callback outputWidth: bus_expand_callback();
      mask Callback outputToWorkspace: bus_expand_callback();
  mult{1..8} (8 alike) : xbsIndex_r4/Mult  precision=User Defined  arith_type="Signed  (2's comp)"  n_bits=36  bin_pt=34  quantization=Truncate  overflow=Wrap  en=off  latency=mult_latency  use_behavioral_HDL=on  opt=Speed  use_embedded=off  optimum_pipeline=off  pipeline=on  dbl_ovrd=off  use_rpm=on  placement_style=Triangular  block_type=mult
  repa : Subsystem  mask(bus_replicate){replication=1, csp_latency=0, misc=off, implementation=core}
      mask prompts: replication "replication factor"; csp_latency "latency"; misc "misc support"; implementation "delay implementation"
      mask help: Output bus formed by replicating input bus a number of times
      mask init:
      | bus_replicate_init(gcb, ...
      |     'replication', replication, ...
      |     'csp_latency', csp_latency, ...
      |     'implementation', implementation, ...
      |     'misc', misc);
      mask TypeOptions implementation: core | behavioral
  repb : Subsystem  mask(bus_replicate){replication=1, csp_latency=0, misc=off, implementation=core}
      mask prompts: replication "replication factor"; csp_latency "latency"; misc "misc support"; implementation "delay implementation"
      mask help: Output bus formed by replicating input bus a number of times
      mask init:
      | bus_replicate_init(gcb, ...
      |     'replication', replication, ...
      |     'csp_latency', csp_latency, ...
      |     'implementation', implementation, ...
      |     'misc', misc);
      mask TypeOptions implementation: core | behavioral
  a*b : Outport
  wires:
  a/1 -> repa/1(in)
  b/1 -> repb/1(in)
  repa/1(out) -> a_debus/1(bus_in)
  repb/1(out) -> b_debus/1(bus_in)
  a_debus/1(msb_out8) -> mult1/1
  b_debus/1(msb_out8) -> mult1/2
  a_debus/2(out7) -> mult2/1
  b_debus/2(out7) -> mult2/2
  a_debus/3(out6) -> mult3/1
  b_debus/3(out6) -> mult3/2
  a_debus/4(out5) -> mult4/1
  b_debus/4(out5) -> mult4/2
  a_debus/5(out4) -> mult5/1
  b_debus/5(out4) -> mult5/2
  a_debus/6(out3) -> mult6/1
  b_debus/6(out3) -> mult6/2
  a_debus/7(out2) -> mult7/1
  b_debus/7(out2) -> mult7/2
  a_debus/8(lsb_out1) -> mult8/1
  b_debus/8(lsb_out1) -> mult8/2
  mult1/1 -> a*b_bussify/1(in1)
  mult2/1 -> a*b_bussify/2(in2)
  mult3/1 -> a*b_bussify/3(in3)
  mult4/1 -> a*b_bussify/4(in4)
  mult5/1 -> a*b_bussify/5(in5)
  mult6/1 -> a*b_bussify/6(in6)
  mult7/1 -> a*b_bussify/7(in7)
  mult8/1 -> a*b_bussify/8(in8)
  a*b_bussify/1(bus_out) -> a*b/1
